simulink model "Rebuilt_Intake_Test"  (R2023b)
settings: Solver=VariableStepAuto  StartTime=0.0  StopTime=inf  MaxStep=0.02  RelTol=1e-3
undefined symbols (not defined in the file or in its folder): RB_Intake_Cycle_Angle_In, RB_Intake_Cycle_Angle_Out, RB_Intake_Des_Angle_In, RB_Intake_Des_Angle_Out
libraries: simulink x1
settings Model: Creator=ander  LastModifiedBy=ander

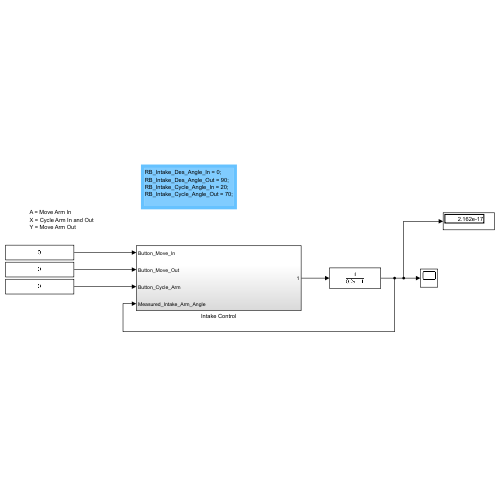
[thumbnail: Simulink's stored preview of the top-level diagram]
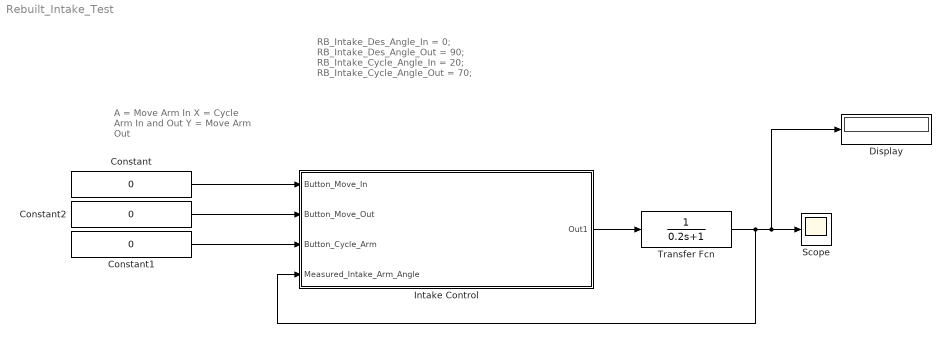
== system Rebuilt_Intake_Test ==
  note: RB_Intake_Des_Angle_In = 0;
      | RB_Intake_Des_Angle_Out = 90;
      | RB_Intake_Cycle_Angle_In = 20;
      | RB_Intake_Cycle_Angle_Out = 70;
  note: A = Move Arm In
      | X = Cycle Arm In and Out
      | Y = Move Arm Out
  Constant : Constant  Value=0  OutDataTypeStr=boolean
  Constant1 : Constant  Value=0  OutDataTypeStr=boolean
  Constant2 : Constant  Value=0  OutDataTypeStr=boolean
  Display : Display
  Intake Control : Subsystem
  Scope : Scope
  Transfer Fcn : TransferFcn  Denominator=[0.2 1]
  wires:
  Constant/1 -> Intake Control/1(Button_Move_In)
  Constant1/1 -> Intake Control/3(Button_Cycle_Arm)
  Constant2/1 -> Intake Control/2(Button_Move_Out)
  Intake Control/1(Out1) -> Transfer Fcn/1
  Transfer Fcn/1 -> Display/1, Scope/1, Intake Control/4(Measured_Intake_Arm_Angle)

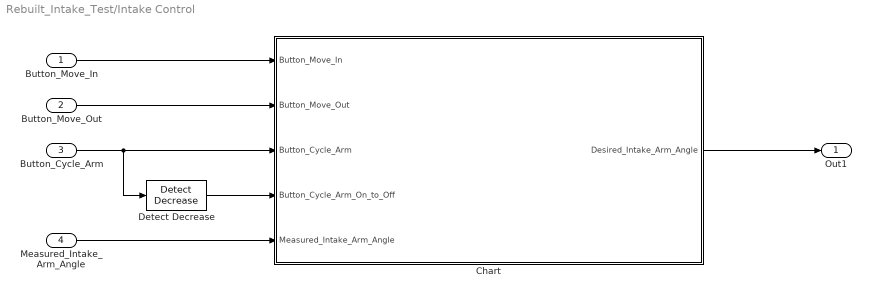
== system Rebuilt_Intake_Test/Intake Control ==
  Button_Move_In : Inport
  Button_Move_Out : Inport  Port=2
  Button_Cycle_Arm : Inport  Port=3
  Measured_Intake_Arm_Angle : Inport  Port=4
  Chart : Stateflow chart  TreatAsAtomicUnit=on
  Detect Decrease : simulink/Logic and Bit Operations/Detect Decrease  vinit=0.0  OutDataTypeStr=boolean
  Out1 : Outport
  wires:
  Button_Move_Out/1 -> Chart/2(Button_Move_Out)
  Button_Move_In/1 -> Chart/1(Button_Move_In)
  Button_Cycle_Arm/1 -> Detect Decrease/1, Chart/3(Button_Cycle_Arm)
  Measured_Intake_Arm_Angle/1 -> Chart/5(Measured_Intake_Arm_Angle)
  Chart/1(Desired_Intake_Arm_Angle) -> Out1/1
  Detect Decrease/1 -> Chart/4(Button_Cycle_Arm_On_to_Off)

== stateflow chart Rebuilt_Intake_Test/Intake Control/Chart ==
  state Wait_for_Button
    entry: Desired_Intake_Arm_Angle = Measured_Intake_Arm_Angle;
  state Move_Intake_Arm_In
    entry: Desired_Intake_Arm_Angle = RB_Intake_Des_Angle_In;
  state Move_Intake_Arm_Out
    entry: Desired_Intake_Arm_Angle = RB_Intake_Des_Angle_Out;
  (default) -> Wait_for_Button
  Wait_for_Button -> Move_Intake_Arm_In [order 1] : [Button_Move_In || ...
      | Button_Cycle_Arm]
  Wait_for_Button -> Move_Intake_Arm_Out [order 2] : [Button_Move_Out || ...
      | Button_Cycle_Arm]
  Move_Intake_Arm_In -> Move_Intake_Arm_Out : [Button_Move_Out || ...
      | (Button_Cycle_Arm && ...
      | Measured_Intake_Arm_Angle < ...
      | RB_Intake_Cycle_Angle_In)]
  Move_Intake_Arm_Out -> Move_Intake_Arm_In : [Button_Move_In || ...
      | (Button_Cycle_Arm && ...
      | Measured_Intake_Arm_Angle > ...
      | RB_Intake_Cycle_Angle_Out) || ...
      | Button_Cycle_Arm_On_to_Off]
  data: Button_Move_In input; Button_Move_Out input; Button_Cycle_Arm input; Button_Cycle_Arm_On_to_Off input; Measured_Intake_Arm_Angle input; Desired_Intake_Arm_Angle output; RB_Intake_Cycle_Angle_In parameter; RB_Intake_Des_Angle_Out parameter; RB_Intake_Des_Angle_In parameter; RB_Intake_Cycle_Angle_Out parameter
